simulink model "PID"  (R2016b)
settings: Solver=VariableStepAuto  StartTime=0.0  StopTime=10  RelTol=1e-3
libraries: simulink x2
settings Model: Creator=Hosein  LastModifiedBy=Hosein

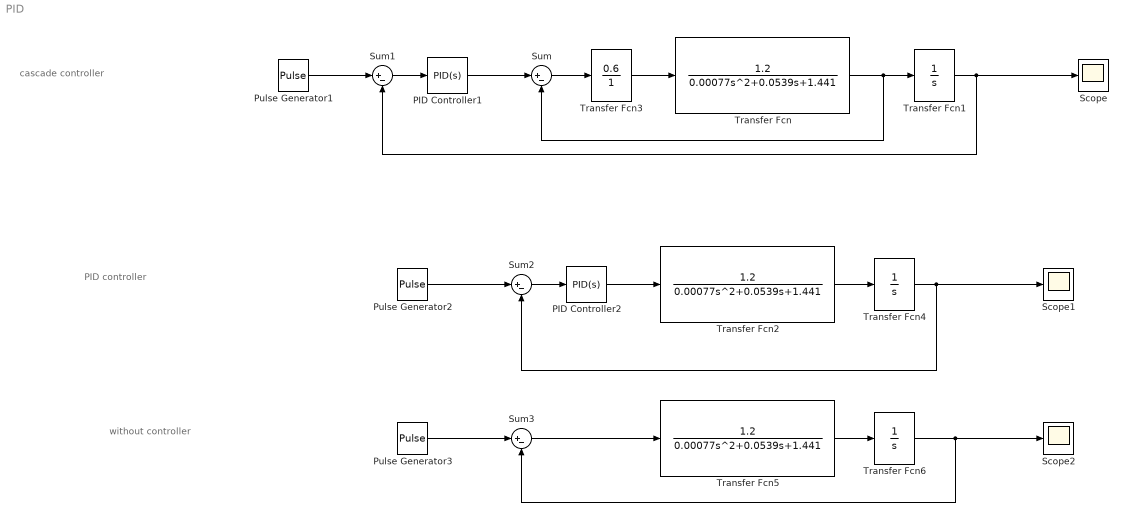
== system PID ==
  note: without controller
  note: PID controller
  note: cascade controller
  PID Controller1 : simulink/Continuous/PID Controller  Controller=PID  TimeDomain=Continuous-time  SampleTime=-1  IntegratorMethod=Forward Euler  FilterMethod=Forward Euler  Form=Parallel  UseFilter=on  ControllerParametersSource=internal  P=63  I=6300/6  D=0.04*63  N=100  InitialConditionSource=internal  InitialConditionForIntegrator=0  InitialConditionForFilter=0  ExternalReset=none  LimitOutput=off  UpperSaturationLimit=inf  LowerSaturationLimit=-inf  LinearizeAsGain=on  AntiWindupMode=none  Kb=1  TrackingMode=off  Kt=1  PParamMin=[]  PParamMax=[]  IParamMin=[]  IParamMax=[]  DParamMin=[]  DParamMax=[]  NParamMin=[]  NParamMax=[]  KbParamMin=[]  KbParamMax=[]  KtParamMin=[]  KtParamMax=[]  POutMin=[]  POutMax=[]  IOutMin=[]  IOutMax=[]  DOutMin=[]  DOutMax=[]  NOutMin=[]  NOutMax=[]  KbOutMin=[]  KbOutMax=[]  KtOutMin=[]  KtOutMax=[]  IntegratorOutMin=[]  IntegratorOutMax=[]  FilterOutMin=[]  FilterOutMax=[]  SumOutMin=[]  SumOutMax=[]  SumI1OutMin=[]  SumI1OutMax=[]  SumI2OutMin=[]  SumI2OutMax=[]  SumI3OutMin=[]  SumI3OutMax=[]  SumDOutMin=[]  SumDOutMax=[]  SaturationOutMin=[]  SaturationOutMax=[]  IntegratorContinuousStateAttributes=''  IntegratorStateMustResolveToSignalObject=off  IntegratorRTWStateStorageClass=Auto  FilterContinuousStateAttributes=''  FilterStateMustResolveToSignalObject=off  FilterRTWStateStorageClass=Auto  DifferentiatorICPrevScaledInput=0  DifferentiatorOutMin=[]  DifferentiatorOutMax=[]
  PID Controller2 : simulink/Continuous/PID Controller  Controller=PID  TimeDomain=Continuous-time  SampleTime=-1  IntegratorMethod=Forward Euler  FilterMethod=Forward Euler  Form=Parallel  UseFilter=on  ControllerParametersSource=internal  P=50.4  I=50.4*14  D=50.4/56  N=100  InitialConditionSource=internal  InitialConditionForIntegrator=0  InitialConditionForFilter=0  ExternalReset=none  LimitOutput=off  UpperSaturationLimit=inf  LowerSaturationLimit=-inf  LinearizeAsGain=on  AntiWindupMode=none  Kb=1  TrackingMode=off  Kt=1  PParamMin=[]  PParamMax=[]  IParamMin=[]  IParamMax=[]  DParamMin=[]  DParamMax=[]  NParamMin=[]  NParamMax=[]  KbParamMin=[]  KbParamMax=[]  KtParamMin=[]  KtParamMax=[]  POutMin=[]  POutMax=[]  IOutMin=[]  IOutMax=[]  DOutMin=[]  DOutMax=[]  NOutMin=[]  NOutMax=[]  KbOutMin=[]  KbOutMax=[]  KtOutMin=[]  KtOutMax=[]  IntegratorOutMin=[]  IntegratorOutMax=[]  FilterOutMin=[]  FilterOutMax=[]  SumOutMin=[]  SumOutMax=[]  SumI1OutMin=[]  SumI1OutMax=[]  SumI2OutMin=[]  SumI2OutMax=[]  SumI3OutMin=[]  SumI3OutMax=[]  SumDOutMin=[]  SumDOutMax=[]  SaturationOutMin=[]  SaturationOutMax=[]  IntegratorContinuousStateAttributes=''  IntegratorStateMustResolveToSignalObject=off  IntegratorRTWStateStorageClass=Auto  FilterContinuousStateAttributes=''  FilterStateMustResolveToSignalObject=off  FilterRTWStateStorageClass=Auto  DifferentiatorICPrevScaledInput=0  DifferentiatorOutMin=[]  DifferentiatorOutMax=[]
  Pulse Generator1 : DiscretePulseGenerator  PulseType=Time based  PulseWidth=0.5
  Pulse Generator2 : DiscretePulseGenerator  PulseType=Time based  PulseWidth=0.5
  Pulse Generator3 : DiscretePulseGenerator  PulseType=Time based  PulseWidth=0.5
  Scope : Scope
  Scope1 : Scope
  Scope2 : Scope
  Sum{,1..3} (4 alike) : Sum  Inputs=|+-
  Transfer Fcn : TransferFcn  Numerator=[1.2]  Denominator=[0.00077 0.0539 1.441]
  Transfer Fcn1 : TransferFcn  Denominator=[1 0]
  Transfer Fcn2 : TransferFcn  Numerator=[1.2]  Denominator=[0.00077 0.0539 1.441]
  Transfer Fcn3 : TransferFcn  Numerator=[0.6]  Denominator=[1]
  Transfer Fcn4 : TransferFcn  Denominator=[1 0]
  Transfer Fcn5 : TransferFcn  Numerator=[1.2]  Denominator=[0.00077 0.0539 1.441]
  Transfer Fcn6 : TransferFcn  Denominator=[1 0]
  wires:
  Transfer Fcn3/1 -> Transfer Fcn/1
  Transfer Fcn/1 -> Sum/2, Transfer Fcn1/1
  Sum/1 -> Transfer Fcn3/1
  PID Controller1/1 -> Sum/1
  Transfer Fcn1/1 -> Sum1/2, Scope/1
  Sum1/1 -> PID Controller1/1
  Pulse Generator1/1 -> Sum1/1
  PID Controller2/1 -> Transfer Fcn2/1
  Transfer Fcn2/1 -> Transfer Fcn4/1
  Sum2/1 -> PID Controller2/1
  Transfer Fcn4/1 -> Scope1/1, Sum2/2
  Pulse Generator2/1 -> Sum2/1
  Transfer Fcn5/1 -> Transfer Fcn6/1
  Sum3/1 -> Transfer Fcn5/1
  Pulse Generator3/1 -> Sum3/1
  Transfer Fcn6/1 -> Sum3/2, Scope2/1
